simulink model "emso"  (Simulink 7.1)
settings: Solver=VariableStepDiscrete  StartTime=0.0  StopTime=360  RelTol=1e-3
settings Model: Creator=lades  LastModifiedBy=lades
settings DataIOCC: ExternalInput=Az

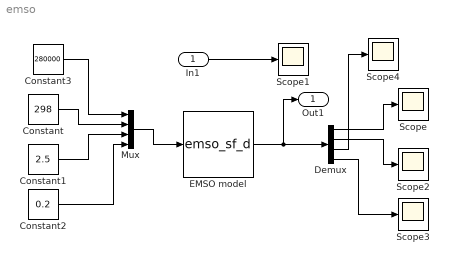
== system emso ==
  In1 : Inport  OutDataType=sfix(16)  OutScaling=2^0
  Constant : Constant  Value=298  OutDataType=sfix(16)  OutScaling=2^0
  Constant1 : Constant  Value=2.5  OutDataType=sfix(16)  OutScaling=2^0
  Constant2 : Constant  Value=0.2  OutDataType=sfix(16)  OutScaling=2^0
  Constant3 : Constant  Value=280000  OutDataType=sfix(16)  OutScaling=2^0
  Demux : Demux
  EMSO model : S-Function  FunctionName=emso_sf_d  Parameters='batch_PID.ems',4,4,0.1  EnableBusSupport=off
  Mux : Mux
  Scope{,1..4} (5 alike) : Scope
      Scope settings: TimeRange=2  YMin=4.008258966500001  YMax=4.008258969500001
      Scope2 settings: TimeRange=2  YMin=4.008258966500001  YMax=4.008258969500001  SaveName=ScopeData2
      Scope3 settings: TimeRange=2  YMin=4.008258966500001  YMax=4.008258969500001  SaveName=ScopeData3
      Scope4 settings: TimeRange=2  YMin=4.008258966500001  YMax=4.008258969500001  SaveName=ScopeData4
  Out1 : Outport  OutDataType=sfix(16)  OutScaling=2^0
  wires:
  EMSO model/1 -> Out1/1, Demux/1
  In1/1 -> Scope1/1
  Constant3/1 -> Mux/1
  Constant/1 -> Mux/2
  Constant1/1 -> Mux/3
  Constant2/1 -> Mux/4
  Mux/1 -> EMSO model/1
  Demux/4 -> Scope3/1
  Demux/3 -> Scope4/1
  Demux/2 -> Scope2/1
  Demux/1 -> Scope/1
